simulink model "single_drone_simulation_R2018b"  (R2018b)
settings: Solver=VariableStepAuto  StartTime=0.0  StopTime=Param.Tend  MaxStep=0.05  MinStep=0.001  RelTol=1e-3
InitFcn:
  | drone_init;
  | iD = 1;
StopFcn:
  | drone_show_data;
undefined symbols (not defined in the file or in its folder): Param
settings Model: SimulationMode=accelerator  Creator=Bruno  LastModifiedBy=Bruno
settings DataIOCC: ReturnWorkspaceOutputs=on
settings DebuggingCC: UnconnectedInputMsg=none  UnconnectedOutputMsg=none  UnconnectedLineMsg=none  SFMachineParentedDataDiag=error
settings ModelReferenceCC: EnableRefExpFcnMdlSchedulingChecks=off
settings RTWCC: Description=Generic Real-Time Target

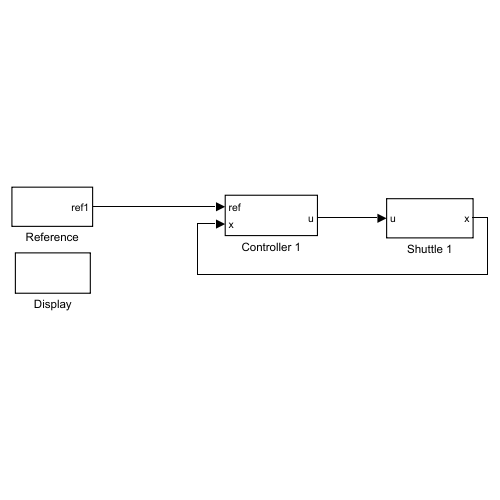
[thumbnail: Simulink's stored preview of the top-level diagram]
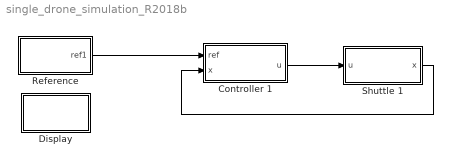
== system single_drone_simulation_R2018b ==
  Controller 1 : Subsystem
  Display : Subsystem
  Reference : Subsystem
  Shuttle 1 : Subsystem
  wires:
  Reference/1(ref1) -> Controller 1/1(ref)
  Shuttle 1/1(x) -> Controller 1/2(x)
  Controller 1/1(u) -> Shuttle 1/1(u)

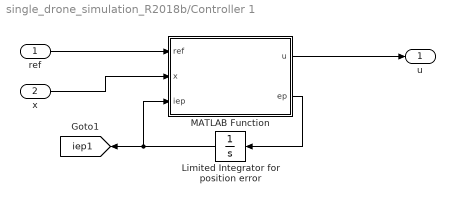
== system single_drone_simulation_R2018b/Controller 1 ==
  ref : Inport
  x : Inport  Port=2
  Limited Integrator for position error : Integrator  LimitOutput=on  UpperSaturationLimit=100  LowerSaturationLimit=-100
  MATLAB Function : MATLAB Function  TreatAsAtomicUnit=on
  u : Outport
  tag scope: iep1=global
  wires:
  MATLAB Function/2(ep) -> Limited Integrator for position error/1
  MATLAB Function/1(u) -> u/1
  Limited Integrator for position error/1 -> [iep1], MATLAB Function/3(iep)
  ref/1 -> MATLAB Function/1(ref)
  x/1 -> MATLAB Function/2(x)

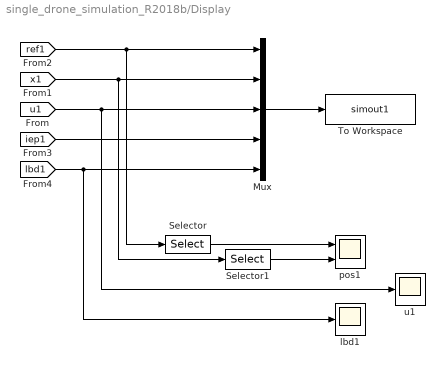
== system single_drone_simulation_R2018b/Display ==
  Mux : Mux  Inputs=5
  Selector : Selector  InputPortWidth=14  IndexOptions=Index vector (dialog)  Indices=[1:3]  OutputSizes=1
  Selector1 : Selector  InputPortWidth=18  IndexOptions=Index vector (dialog)  Indices=[1:3]  OutputSizes=1
  To Workspace : ToWorkspace  VariableName=simout1  SaveFormat=Structure With Time  SampleTime=-1
  lbd1 : Scope
  pos1 : Scope  NumInputPorts=2
  u1 : Scope
  wires:
  [x1] -> Selector1/1, Mux/2
  [u1] -> u1/1, Mux/3
  [iep1] -> Mux/4
  [ref1] -> Selector/1, Mux/1
  Mux/1 -> To Workspace/1
  Selector/1 -> pos1/1
  Selector1/1 -> pos1/2
  [lbd1] -> lbd1/1, Mux/5

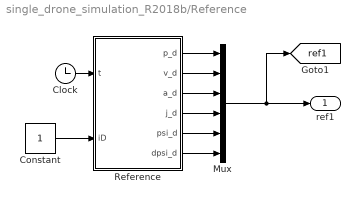
== system single_drone_simulation_R2018b/Reference ==
  Clock : Clock
  Constant : Constant
  Mux : Mux  Inputs=6
  Reference : MATLAB Function  TreatAsAtomicUnit=on
  ref1 : Outport
  tag scope: ref1=global
  wires:
  Reference/5(psi_d) -> Mux/5
  Reference/3(a_d) -> Mux/3
  Clock/1 -> Reference/1(t)
  Mux/1 -> [ref1], ref1/1
  Reference/1(p_d) -> Mux/1
  Reference/2(v_d) -> Mux/2
  Reference/4(j_d) -> Mux/4
  Reference/6(dpsi_d) -> Mux/6
  Constant/1 -> Reference/2(iD)

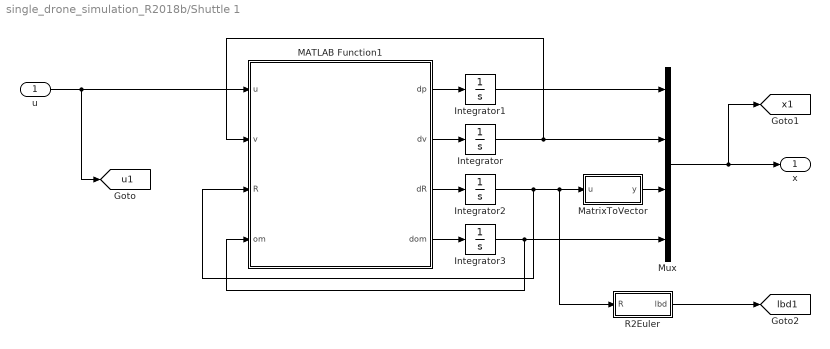
== system single_drone_simulation_R2018b/Shuttle 1 ==
  u : Inport
  Integrator : Integrator  InitialCondition=Param.v0_1  ContinuousStateAttributes='v'
  Integrator1 : Integrator  InitialCondition=Param.p0_1  ContinuousStateAttributes='p'
  Integrator2 : Integrator  InitialCondition=Param.R0_1  ContinuousStateAttributes='R'
  Integrator3 : Integrator  InitialCondition=Param.om0_1  ContinuousStateAttributes='om'
  MATLAB Function1 : MATLAB Function  TreatAsAtomicUnit=on
  MatrixToVector : MATLAB Function  TreatAsAtomicUnit=on
  Mux : Mux
  R2Euler : MATLAB Function  TreatAsAtomicUnit=on
  x : Outport
  tag scope: lbd1=global, u1=global, x1=global
  wires:
  Integrator/1 -> MATLAB Function1/2(v), Mux/2
  Integrator2/1 -> MATLAB Function1/3(R), R2Euler/1(R), MatrixToVector/1(u)
  MATLAB Function1/4(dom) -> Integrator3/1
  MATLAB Function1/2(dv) -> Integrator/1
  MATLAB Function1/3(dR) -> Integrator2/1
  MatrixToVector/1(y) -> Mux/3
  Integrator3/1 -> MATLAB Function1/4(om), Mux/4
  Integrator1/1 -> Mux/1
  MATLAB Function1/1(dp) -> Integrator1/1
  u/1 -> [u1], MATLAB Function1/1(u)
  Mux/1 -> [x1], x/1
  R2Euler/1(lbd) -> [lbd1]

== matlab function single_drone_simulation_R2018b/Controller 1/MATLAB Function ==
  data: ref input; x input; iep input size=3; u output size=4; Param parameter; ep output
function [u,ep] = controller(ref,x,iep,Param)
    
    p = x(1:3,1);
    v = x(4:6,1);
    R = reshape(x(7:15,1),3,3);
    om = x(16:18,1);

    p_d = ref(1:3,1);
    v_d = ref(4:6,1);
    a_d = ref(7:9,1);
    j_d = ref(10:12,1);
    psi_d = ref(13,1);
    dpsi_d = ref(14,1);

    [T,tau,ep] = drone_mellinger_ctrl(p,v,R,om,Param,p_d,psi_d,iep,v_d,dpsi_d,a_d,j_d);

    u = [T;tau];
    
end

== matlab function single_drone_simulation_R2018b/Reference/Reference ==
  data: t input; iD input; p_d output; v_d output; a_d output; j_d output; psi_d output; dpsi_d output; Param parameter
function [p_d,v_d,a_d,j_d,psi_d,dpsi_d] = get_ref(t,iD,Param)
    
    [p_d,v_d,a_d,j_d,psi_d,dpsi_d] = gen_reference(t,iD,Param);

end

== matlab function single_drone_simulation_R2018b/Shuttle 1/MATLAB Function1 ==
  data: u input; dp output; v input; R input; om input; dv output; dR output; dom output; Param parameter
function [dp,dv,dR,dom] = dynamics(u,v,R,om,Param)
        
    T = u(1,1);
    tau = u(2:4,1);
    [dp,dv,dR,dom] = drone_3dfull_dyn(v,R,om,T,tau,Param);
    
end

== matlab function single_drone_simulation_R2018b/Shuttle 1/MatrixToVector ==
  data: u input; y output
function y = fcn(u)

y = u(:);

== matlab function single_drone_simulation_R2018b/Shuttle 1/R2Euler ==
  data: R input; lbd output
function lbd = fcn(R)

lbd = R2Euler(R);
